simulink model "TB24_StageA_ModuleFault"  (R2025a)
settings: Solver=FixedStepDiscrete  StartTime=0  StopTime=TB.t_end  FixedStep=TB.dt  RelTol=1e-3
InitFcn:
  | % 모델과 같은 폴더의 초기화 스크립트를 실행해 P(설계 파라미터)와 TB(시험 조건)를 만든다.
  | run(fullfile(fileparts(get_param(bdroot, 'FileName')), 'TB24_init.m'));
values from neighbouring files (symbols this model uses):
  TB = struct()    [TB24_init.m]    (also in run_TB24.m = evalin('base', 'TB'))
libraries: fl_lib x126, nesl_utility x55
(part 1 of 3)
settings Model: Creator=hj000  LastModifiedBy=hj000
settings DataIOCC: SaveOutput=off  SignalLogging=off  SaveTime=off

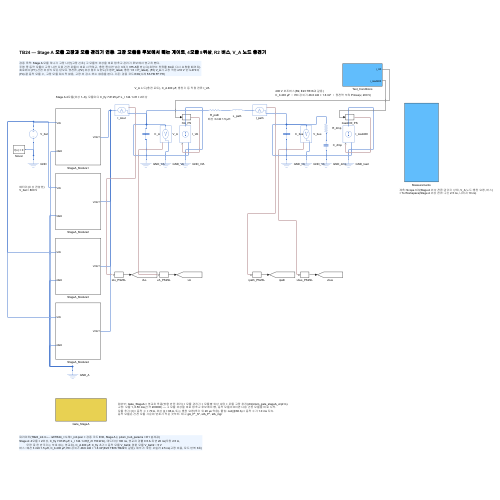
[thumbnail: Simulink's stored preview of the top-level diagram]
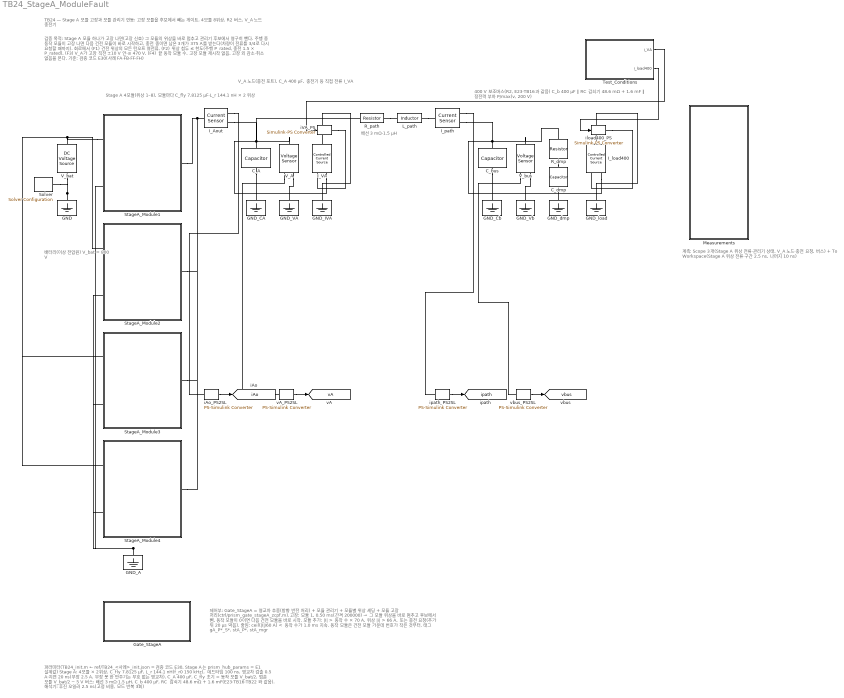
== system TB24_StageA_ModuleFault ==
  note: TB24 — Stage A 모듈 고장과 모듈 관리기 연동: 고장 모듈을 후보에서 빼는 게이트, 4모듈 8위상, R2 버스, V_A 노드 충전기
  note: 검증 목적: Stage A 모듈 하나가 고장 나면(고장 신호) 그 모듈의 위상을 바로 멈추고 관리기 후보에서 영구히 뺀다.
      | 주행 중 동작 모듈이 고장 나면 다음 건전 모듈이 바로 시작하고, 충전 중이면 남은 3개가 375 A를 받는다(차량이 전류를 3/4로 다시 요청할 때까지).
      | 회로에서 (F1) 건전 위상의 모든 턴오프 영전류, (F2) 위상 첨두 ≤ 한도(주행 P_rated, 충전 1.5 × P_rated), (F3) V_A가 고장 직전 ±10 V 안·≤ 470 V,
      | (F4) 끝 동작 모듈 수, 고장 모듈 재시작 없음, 고장 외 감소·취소 없음을 본다. 기준: 검증 코드 E30(사례 FA·FB·FF·FH)
  note: 배터리(이상 전압원)
      | V_bat = 800 V
  note: Stage A 4모듈(위상 1–8), 모듈마다 C_fly 7.8125 µF·L_r 144.1 nH × 2위상
  note: V_A 노드(충전 포트), C_A 400 µF, 충전기 등 직접 전류 I_VA
  note: 배선 3 mΩ·1.5 µH
  note: 400 V 보조버스(R2, E23·TB16과 같음)
      | C_b 400 µF ∥ RC 감쇠기 48.6 mΩ + 1.6 mF ∥ 정전력 부하 P/max(v, 200 V)
  note: 제어부: Gate_StageA = 영교차 추종(방향 반전 처리) + 모듈 관리기 + 모듈별 위상 셰딩 + 모듈 고장 처리(ctrl/prism_gate_stageA_zcpf.m).
      | 고장: 모듈 1, 0.50 ms(간격 200000) → 그 모듈 위상을 바로 멈추고 후보에서 뺌, 동작 모듈이 0이면 다음 건전 모듈을 바로 시작.
      | 모듈 추가: |I| > 동작 수 × 70 A, 위상 |i| > 66 A, 또는 충전 요청(추가 뒤 20 µs 막음). 줄임: ceil(|I|/60 A) < 동작 수가 1.0 ms 지속.
      | 동작 모듈은 건전 모듈 가운데 번호가 작은 것부터. 태그 gA_P*_S*, stA_P*, stA_mgr
  note: 계측: Scope 3개(Stage A 위상 전류·관리기 상태, V_A 노드·충전 요청, 버스)
      | + To Workspace(Stage A 위상 전류·구간 2.5 ns, 나머지 10 ns)
  note: 파라미터(TB24_init.m ← ref/TB24_<사례>_init.json = 검증 코드 E30, Stage A는 prism_hub_params = E1 설계값)
      | Stage A: 4모듈 × 2위상, C_fly 7.8125 µF, L_r 144.1 nH(f_r0 150 kHz), 데드타임 100 ns, 영교차 검출 0.5 A·지연 20 ns(무장 2.5 A,
      |          무장 못 한 반주기는 부호 없는 영교차), C_A 400 µF, C_fly 초기 = 동작 모듈 V_bat/2, 멈춘 모듈 V_bat/2 − 5 V
      | 버스: 배선 3 mΩ·1.5 µH, C_b 400 µF, RC 감쇠기 48.6 mΩ + 1.6 mF(E23·TB16·TB22와 같음). 해석기: 후진 오일러 2.5 ns(고정 비용, 모드 반복 3회)
  C_A : fl_lib/Electrical/Electrical Elements/Capacitor  c=TB.A.CA F  r=1e-6 Ohm  g=0 1/Ohm  i_specify=off  i_priority=None  i=0 A  i_nominal_specify=off  i_nominal_value=1  i_nominal_unit=A  v_specify=off  v_priority=None  v=0 V  v_nominal_specify=off  v_nominal_value=1  v_nominal_unit=V  vc_specify=on  vc_priority=High  vc=TB.vA0 V  vc_nominal_specify=off  vc_nominal_value=1  vc_nominal_unit=V
  C_bus : fl_lib/Electrical/Electrical Elements/Capacitor  c=TB.Cb F  r=1e-6 Ohm  g=0 1/Ohm  i_specify=off  i_priority=None  i=0 A  i_nominal_specify=off  i_nominal_value=1  i_nominal_unit=A  v_specify=off  v_priority=None  v=0 V  v_nominal_specify=off  v_nominal_value=1  v_nominal_unit=V  vc_specify=on  vc_priority=High  vc=TB.vb0 V  vc_nominal_specify=off  vc_nominal_value=1  vc_nominal_unit=V
  C_dmp : fl_lib/Electrical/Electrical Elements/Capacitor  c=TB.Cdmp F  r=1e-6 Ohm  g=0 1/Ohm  i_specify=off  i_priority=None  i=0 A  i_nominal_specify=off  i_nominal_value=1  i_nominal_unit=A  v_specify=off  v_priority=None  v=0 V  v_nominal_specify=off  v_nominal_value=1  v_nominal_unit=V  vc_specify=on  vc_priority=High  vc=TB.vb0 V  vc_nominal_specify=off  vc_nominal_value=1  vc_nominal_unit=V
  GND : fl_lib/Electrical/Electrical Elements/Electrical Reference
  GND_A : fl_lib/Electrical/Electrical Elements/Electrical Reference
  GND_CA : fl_lib/Electrical/Electrical Elements/Electrical Reference
  GND_Cb : fl_lib/Electrical/Electrical Elements/Electrical Reference
  GND_IVA : fl_lib/Electrical/Electrical Elements/Electrical Reference
  GND_VA : fl_lib/Electrical/Electrical Elements/Electrical Reference
  GND_Vb : fl_lib/Electrical/Electrical Elements/Electrical Reference
  GND_dmp : fl_lib/Electrical/Electrical Elements/Electrical Reference
  GND_load : fl_lib/Electrical/Electrical Elements/Electrical Reference
  Gate_StageA : Subsystem
  I_Aout : fl_lib/Electrical/Electrical Sensors/Current Sensor
  I_VA : fl_lib/Electrical/Electrical Sources/Controlled Current Source
  I_load400 : fl_lib/Electrical/Electrical Sources/Controlled Current Source
  I_path : fl_lib/Electrical/Electrical Sensors/Current Sensor
  L_path : fl_lib/Electrical/Electrical Elements/Inductor  l=TB.Lpath H  r=0 Ohm  g=1e-9 1/Ohm  i_specify=off  i_priority=None  i=0 A  i_nominal_specify=off  i_nominal_value=1  i_nominal_unit=A  v_specify=off  v_priority=None  v=0 V  v_nominal_specify=off  v_nominal_value=1  v_nominal_unit=V  i_L_specify=on  i_L_priority=High  i_L=TB.iw0 A  i_L_nominal_specify=off  i_L_nominal_value=1  i_L_nominal_unit=A
  Measurements : Subsystem
  R_dmp : fl_lib/Electrical/Electrical Elements/Resistor  R=TB.Rdmp Ohm  i_specify=off  i_priority=None  i=0 A  i_nominal_specify=off  i_nominal_value=1  i_nominal_unit=A  v_specify=off  v_priority=None  v=0 V  v_nominal_specify=off  v_nominal_value=1  v_nominal_unit=V
  R_path : fl_lib/Electrical/Electrical Elements/Resistor  R=TB.Rpath Ohm  i_specify=off  i_priority=None  i=0 A  i_nominal_specify=off  i_nominal_value=1  i_nominal_unit=A  v_specify=off  v_priority=None  v=0 V  v_nominal_specify=off  v_nominal_value=1  v_nominal_unit=V
  Solver : nesl_utility/Solver Configuration  PhysicalDomain=network_engine_domain  SubClassName=solver  LeftPortType=input  RightPortType=generic  Tones=[]  Harmonics=[]  SimulateNoise=off  Profile=off  UseLocalSampling=off  EnableSwitchedLinearOptims=on  FrequencyDomain=off  UseCCode=off  RelTol=0.001  AbsTol=0.001  MinStep=1e-09  ToWorkspace=off  RevertToSquareIcSolve=off  NumHomotopyIterations=100  PhasorMode=off  PhasorModeNumHarmonics=1  ConsistencySolver=NEWTON_XTOL_AFTER_FTOL  IndexReductionMethod=DerivativeReplacement  DoDC=off  ResidualTolerance=1e-9  ConsistencyTolSource=GLOBAL  ConsistencyAbsTol=0.001  ConsistencyRelTol=0.001  ConsistencyTolFactor=0.001  UseLocalSolver=on  LocalSolverChoice=NE_BACKWARD_EULER_ADVANCER  ResolveIndetEquations=on  FunctionEvalNumThread=1  LocalSolverSampleTime=TB.dt  DoFixedCost=on  MaxNonlinIter=3  MaxModeIter=2  ComputeImpulses=off  ImpulseIterations=2  LinearAlgebra=auto  LinearAlgebraNumThread=0  EquationFormulation=NE_TIME_EF  DelaysMemoryBudget=1024  AutomaticFiltering=on  FilteringTimeConstant=0.001  PartitionStorageMethod=AS_NEEDED  PartitionMemoryBudget=1024  PartitionMethod=ROBUST  MultibodyUseLocalSolver=off  MultibodyLocalSolverChoice=ODE1  MultibodyLocalSolverSampleTime=0.001
  StageA_Module1 : Subsystem
  StageA_Module2 : Subsystem
  StageA_Module3 : Subsystem
  StageA_Module4 : Subsystem
  Test_Conditions : Subsystem
  V_A : fl_lib/Electrical/Electrical Sensors/Voltage Sensor
  V_bat : fl_lib/Electrical/Electrical Sources/DC Voltage Source  v0=TB.vbat V
  V_bus : fl_lib/Electrical/Electrical Sensors/Voltage Sensor
  iAo_PS2SL : nesl_utility/PS-Simulink Converter  PhysicalDomain=network_engine_domain  SubClassName=ps_output  LeftPortType=input  RightPortType=output  PseudoPeriodic=off  Frequencies=[]  VectorFormat=inherit  Unit=inherit  AffineConversion=off
  iVA_PS : nesl_utility/Simulink-PS Converter  PhysicalDomain=network_engine_domain  SubClassName=ps_input  LeftPortType=input  RightPortType=output  PseudoPeriodic=off  Frequencies=[]  NoiseDistribution=none  NoiseParameters=[]  Unit=1  AffineConversion=off  FilteringAndDerivatives=provide  SimscapeFilterOrder=1  InputFilterTimeConstant=0.001  UdotUserProvided=0
  iload400_PS : nesl_utility/Simulink-PS Converter  PhysicalDomain=network_engine_domain  SubClassName=ps_input  LeftPortType=input  RightPortType=output  PseudoPeriodic=off  Frequencies=[]  NoiseDistribution=none  NoiseParameters=[]  Unit=1  AffineConversion=off  FilteringAndDerivatives=provide  SimscapeFilterOrder=1  InputFilterTimeConstant=0.001  UdotUserProvided=0
  ipath_PS2SL : nesl_utility/PS-Simulink Converter  PhysicalDomain=network_engine_domain  SubClassName=ps_output  LeftPortType=input  RightPortType=output  PseudoPeriodic=off  Frequencies=[]  VectorFormat=inherit  Unit=inherit  AffineConversion=off
  vA_PS2SL : nesl_utility/PS-Simulink Converter  PhysicalDomain=network_engine_domain  SubClassName=ps_output  LeftPortType=input  RightPortType=output  PseudoPeriodic=off  Frequencies=[]  VectorFormat=inherit  Unit=inherit  AffineConversion=off
  vbus_PS2SL : nesl_utility/PS-Simulink Converter  PhysicalDomain=network_engine_domain  SubClassName=ps_output  LeftPortType=input  RightPortType=output  PseudoPeriodic=off  Frequencies=[]  VectorFormat=inherit  Unit=inherit  AffineConversion=off
  tag scope: iAo=global, ipath=global, vA=global, vbus=global
  wires:
  iAo_PS2SL/1 -> [iAo]
  vA_PS2SL/1 -> [vA]
  ipath_PS2SL/1 -> [ipath]
  vbus_PS2SL/1 -> [vbus]
  Test_Conditions/1(i_VA) -> iVA_PS/1
  Test_Conditions/2(i_load400) -> iload400_PS/1
  connections:
  GND/LConn1 -- Solver/RConn1 -- V_bat/RConn1
  StageA_Module1/LConn1 -- V_bat/LConn1 -- StageA_Module2/LConn1 -- StageA_Module3/LConn1 -- StageA_Module4/LConn1
  StageA_Module1/LConn2 -- StageA_Module2/LConn2 -- StageA_Module3/LConn2 -- GND_A/LConn1 -- StageA_Module4/LConn2
  StageA_Module1/RConn1 -- StageA_Module2/RConn1 -- StageA_Module3/RConn1 -- I_Aout/LConn1 -- StageA_Module4/RConn1
  I_Aout/RConn2 -- V_A/LConn1 -- I_VA/RConn2 -- C_A/LConn1 -- R_path/LConn1
  C_A/RConn1 -- GND_CA/LConn1
  V_A/RConn2 -- GND_VA/LConn1
  I_VA/LConn1 -- GND_IVA/LConn1
  iVA_PS/RConn1 -- I_VA/RConn1
  R_path/RConn1 -- L_path/LConn1
  L_path/RConn1 -- I_path/LConn1
  I_path/RConn2 -- V_bus/LConn1 -- R_dmp/LConn1 -- C_bus/LConn1 -- I_load400/RConn2
  C_bus/RConn1 -- GND_Cb/LConn1
  V_bus/RConn2 -- GND_Vb/LConn1
  R_dmp/RConn1 -- C_dmp/LConn1
  C_dmp/RConn1 -- GND_dmp/LConn1
  I_load400/LConn1 -- GND_load/LConn1
  iload400_PS/RConn1 -- I_load400/RConn1
  I_Aout/RConn1 -- iAo_PS2SL/LConn1
  V_A/RConn1 -- vA_PS2SL/LConn1
  I_path/RConn1 -- ipath_PS2SL/LConn1
  V_bus/RConn1 -- vbus_PS2SL/LConn1

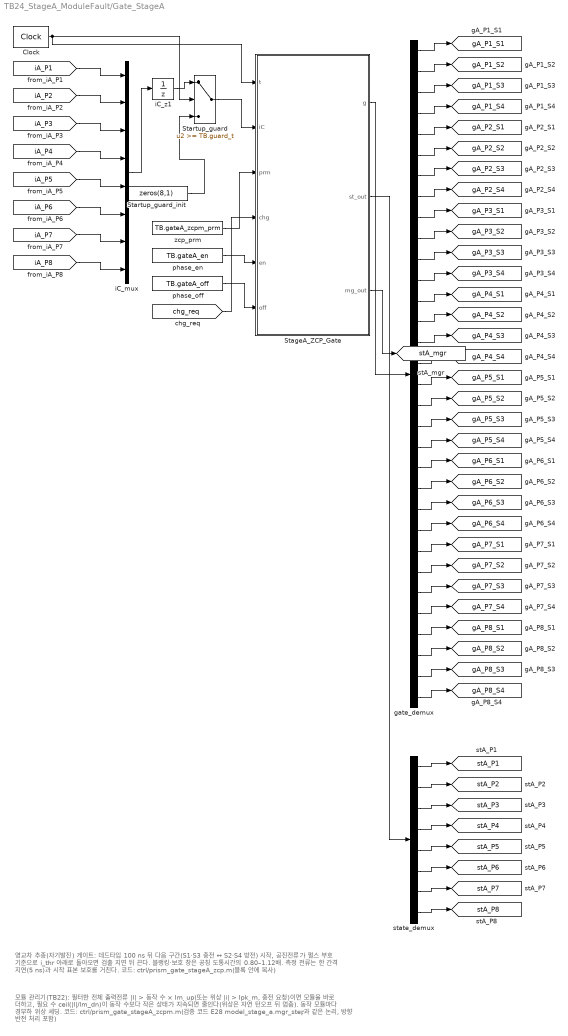
== system TB24_StageA_ModuleFault/Gate_StageA ==
  note: 모듈 관리기(TB22): 필터한 전체 출력전류 |I| > 동작 수 × Im_up(또는 위상 |i| > Ipk_m, 충전 요청)이면 모듈을 바로 더하고,
      | 필요 수 ceil(|I|/Im_dn)이 동작 수보다 작은 상태가 지속되면 줄인다(위상은 자연 턴오프 뒤 멈춤). 동작 모듈마다 경부하 위상 셰딩.
      | 코드: ctrl/prism_gate_stageA_zcpm.m(검증 코드 E28 model_stage_a.mgr_step과 같은 논리, 방향 반전 처리 포함)
  note: 영교차 추종(자기발진) 게이트: 데드타임 100 ns 뒤 다음 구간(S1·S3 충전 ↔ S2·S4 방전) 시작,
      | 공진전류가 펄스 부호 기준으로 i_thr 아래로 돌아오면 검출 지연 뒤 끈다. 블랭킹·보호 창은 공칭 도통시간의 0.80–1.12배.
      | 측정 전류는 한 간격 지연(5 ns)과 시작 표본 보호를 거친다. 코드: ctrl/prism_gate_stageA_zcp.m(블록 안에 복사)
  Clock : DigitalClock  SampleTime=TB.dt
  StageA_ZCP_Gate : MATLAB Function  TreatAsAtomicUnit=on
  Startup_guard : Switch  Threshold=TB.guard_t  SaturateOnIntegerOverflow=off  InputSameDT=off
  Startup_guard_init : Constant  Value=zeros(8,1)
  gate_demux : Demux  Outputs=[1 1 1 1 1 1 1 1 1 1 1 1 1 1 1 1 1 1 1 1 1 1 1 1 1 1 1 1 1 1 1 1]
  iC_mux : Mux  Inputs=8
  iC_z1 : UnitDelay  SampleTime=TB.dt  HasFrameUpgradeWarning=on
  phase_en : Constant  Value=TB.gateA_en
  phase_off : Constant  Value=TB.gateA_off
  state_demux : Demux  Outputs=[1 1 1 1 1 1 1 1]
  zcp_prm : Constant  Value=TB.gateA_zcpm_prm
  tag scope: gA_P1_S1=global, gA_P1_S2=global, gA_P1_S3=global, gA_P1_S4=global, gA_P2_S1=global, gA_P2_S2=global, gA_P2_S3=global, gA_P2_S4=global, gA_P3_S1=global, gA_P3_S2=global, gA_P3_S3=global, gA_P3_S4=global, gA_P4_S1=global, gA_P4_S2=global, gA_P4_S3=global, gA_P4_S4=global, gA_P5_S1=global, gA_P5_S2=global, gA_P5_S3=global, gA_P5_S4=global, gA_P6_S1=global, gA_P6_S2=global, gA_P6_S3=global, gA_P6_S4=global, gA_P7_S1=global, gA_P7_S2=global, gA_P7_S3=global, gA_P7_S4=global, gA_P8_S1=global, gA_P8_S2=global, gA_P8_S3=global, gA_P8_S4=global, stA_P1=global, stA_P2=global, stA_P3=global, stA_P4=global, stA_P5=global, stA_P6=global, stA_P7=global, stA_P8=global, stA_mgr=global
  wires:
  [iA_P1] -> iC_mux/1
  [iA_P2] -> iC_mux/2
  [iA_P3] -> iC_mux/3
  [iA_P4] -> iC_mux/4
  [iA_P5] -> iC_mux/5
  [iA_P6] -> iC_mux/6
  [iA_P7] -> iC_mux/7
  [iA_P8] -> iC_mux/8
  iC_mux/1 -> iC_z1/1
  Startup_guard_init/1 -> Startup_guard/3
  iC_z1/1 -> Startup_guard/1
  Clock/1 -> Startup_guard/2, StageA_ZCP_Gate/1(t)
  StageA_ZCP_Gate/3(mg_out) -> [stA_mgr]
  Startup_guard/1 -> StageA_ZCP_Gate/2(iC)
  zcp_prm/1 -> StageA_ZCP_Gate/3(prm)
  [chg_req] -> StageA_ZCP_Gate/4(chg)
  phase_en/1 -> StageA_ZCP_Gate/5(en)
  phase_off/1 -> StageA_ZCP_Gate/6(off)
  StageA_ZCP_Gate/1(g) -> gate_demux/1
  gate_demux/1 -> [gA_P1_S1]
  gate_demux/2 -> [gA_P1_S2]
  gate_demux/3 -> [gA_P1_S3]
  gate_demux/4 -> [gA_P1_S4]
  gate_demux/5 -> [gA_P2_S1]
  gate_demux/6 -> [gA_P2_S2]
  gate_demux/7 -> [gA_P2_S3]
  gate_demux/8 -> [gA_P2_S4]
  gate_demux/9 -> [gA_P3_S1]
  gate_demux/10 -> [gA_P3_S2]
  gate_demux/11 -> [gA_P3_S3]
  gate_demux/12 -> [gA_P3_S4]
  gate_demux/13 -> [gA_P4_S1]
  gate_demux/14 -> [gA_P4_S2]
  gate_demux/15 -> [gA_P4_S3]
  gate_demux/16 -> [gA_P4_S4]
  gate_demux/17 -> [gA_P5_S1]
  gate_demux/18 -> [gA_P5_S2]
  gate_demux/19 -> [gA_P5_S3]
  gate_demux/20 -> [gA_P5_S4]
  gate_demux/21 -> [gA_P6_S1]
  gate_demux/22 -> [gA_P6_S2]
  gate_demux/23 -> [gA_P6_S3]
  gate_demux/24 -> [gA_P6_S4]
  gate_demux/25 -> [gA_P7_S1]
  gate_demux/26 -> [gA_P7_S2]
  gate_demux/27 -> [gA_P7_S3]
  gate_demux/28 -> [gA_P7_S4]
  gate_demux/29 -> [gA_P8_S1]
  gate_demux/30 -> [gA_P8_S2]
  gate_demux/31 -> [gA_P8_S3]
  gate_demux/32 -> [gA_P8_S4]
  StageA_ZCP_Gate/2(st_out) -> state_demux/1
  state_demux/1 -> [stA_P1]
  state_demux/2 -> [stA_P2]
  state_demux/3 -> [stA_P3]
  state_demux/4 -> [stA_P4]
  state_demux/5 -> [stA_P5]
  state_demux/6 -> [stA_P6]
  state_demux/7 -> [stA_P7]
  state_demux/8 -> [stA_P8]

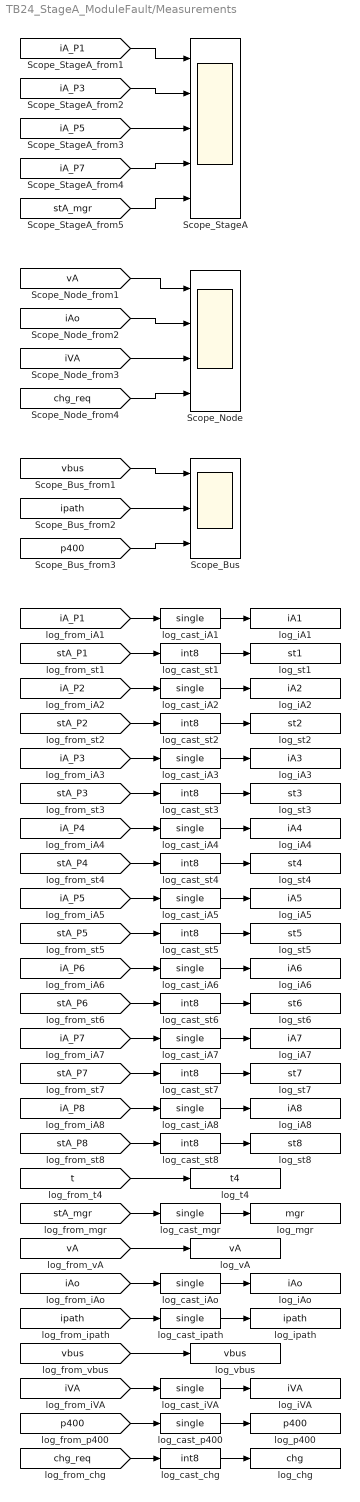
== system TB24_StageA_ModuleFault/Measurements ==
  Scope_Bus : Scope  NumInputPorts=3
      settings: Title=Scope Bus
  Scope_Node : Scope  NumInputPorts=4
      settings: Title=Scope Node
  Scope_StageA : Scope  NumInputPorts=5
      settings: Title=Scope StageA
  log_cast_chg : DataTypeConversion  OutDataTypeStr=int8  SaturateOnIntegerOverflow=off  RndMeth=Floor
  log_cast_iA{1..8} (8 alike) : DataTypeConversion  OutDataTypeStr=single  SaturateOnIntegerOverflow=off  RndMeth=Floor
  log_cast_iAo : DataTypeConversion  OutDataTypeStr=single  SaturateOnIntegerOverflow=off  RndMeth=Floor
  log_cast_iVA : DataTypeConversion  OutDataTypeStr=single  SaturateOnIntegerOverflow=off  RndMeth=Floor
  log_cast_ipath : DataTypeConversion  OutDataTypeStr=single  SaturateOnIntegerOverflow=off  RndMeth=Floor
  log_cast_mgr : DataTypeConversion  OutDataTypeStr=single  SaturateOnIntegerOverflow=off  RndMeth=Floor
  log_cast_p400 : DataTypeConversion  OutDataTypeStr=single  SaturateOnIntegerOverflow=off  RndMeth=Floor
  log_cast_st{1..8} (8 alike) : DataTypeConversion  OutDataTypeStr=int8  SaturateOnIntegerOverflow=off  RndMeth=Floor
  log_chg : ToWorkspace  VariableName=chg  SampleTime=-1
      settings: Decimation=4
  log_iA1 : ToWorkspace  VariableName=iA1  SampleTime=-1
  log_iA2 : ToWorkspace  VariableName=iA2  SampleTime=-1
  log_iA3 : ToWorkspace  VariableName=iA3  SampleTime=-1
  log_iA4 : ToWorkspace  VariableName=iA4  SampleTime=-1
  log_iA5 : ToWorkspace  VariableName=iA5  SampleTime=-1
  log_iA6 : ToWorkspace  VariableName=iA6  SampleTime=-1
  log_iA7 : ToWorkspace  VariableName=iA7  SampleTime=-1
  log_iA8 : ToWorkspace  VariableName=iA8  SampleTime=-1
  log_iAo : ToWorkspace  VariableName=iAo  SampleTime=-1
      settings: Decimation=4
  log_iVA : ToWorkspace  VariableName=iVA  SampleTime=-1
      settings: Decimation=4
  log_ipath : ToWorkspace  VariableName=ipath  SampleTime=-1
      settings: Decimation=4
  log_mgr : ToWorkspace  VariableName=mgr  SampleTime=-1
      settings: Decimation=4
  log_p400 : ToWorkspace  VariableName=p400  SampleTime=-1
      settings: Decimation=4
  log_st1 : ToWorkspace  VariableName=st1  SampleTime=-1
  log_st2 : ToWorkspace  VariableName=st2  SampleTime=-1
  log_st3 : ToWorkspace  VariableName=st3  SampleTime=-1
  log_st4 : ToWorkspace  VariableName=st4  SampleTime=-1
  log_st5 : ToWorkspace  VariableName=st5  SampleTime=-1
  log_st6 : ToWorkspace  VariableName=st6  SampleTime=-1
  log_st7 : ToWorkspace  VariableName=st7  SampleTime=-1
  log_st8 : ToWorkspace  VariableName=st8  SampleTime=-1
  log_t4 : ToWorkspace  VariableName=t4  SampleTime=-1
      settings: Decimation=4
  log_vA : ToWorkspace  VariableName=vA  SampleTime=-1
      settings: Decimation=4
  log_vbus : ToWorkspace  VariableName=vbus  SampleTime=-1
      settings: Decimation=4
  wires:
  [iA_P1] -> Scope_StageA/1
  [iA_P3] -> Scope_StageA/2
  [iA_P5] -> Scope_StageA/3
  [iA_P7] -> Scope_StageA/4
  [stA_mgr] -> Scope_StageA/5
  [vA] -> Scope_Node/1
  [iAo] -> Scope_Node/2
  [iVA] -> Scope_Node/3
  [chg_req] -> Scope_Node/4
  [vbus] -> Scope_Bus/1
  [ipath] -> Scope_Bus/2
  [p400] -> Scope_Bus/3
  [iA_P1] -> log_cast_iA1/1
  log_cast_iA1/1 -> log_iA1/1
  [stA_P1] -> log_cast_st1/1
  log_cast_st1/1 -> log_st1/1
  [iA_P2] -> log_cast_iA2/1
  log_cast_iA2/1 -> log_iA2/1
  [stA_P2] -> log_cast_st2/1
  log_cast_st2/1 -> log_st2/1
  [iA_P3] -> log_cast_iA3/1
  log_cast_iA3/1 -> log_iA3/1
  [stA_P3] -> log_cast_st3/1
  log_cast_st3/1 -> log_st3/1
  [iA_P4] -> log_cast_iA4/1
  log_cast_iA4/1 -> log_iA4/1
  [stA_P4] -> log_cast_st4/1
  log_cast_st4/1 -> log_st4/1
  [iA_P5] -> log_cast_iA5/1
  log_cast_iA5/1 -> log_iA5/1
  [stA_P5] -> log_cast_st5/1
  log_cast_st5/1 -> log_st5/1
  [iA_P6] -> log_cast_iA6/1
  log_cast_iA6/1 -> log_iA6/1
  [stA_P6] -> log_cast_st6/1
  log_cast_st6/1 -> log_st6/1
  [iA_P7] -> log_cast_iA7/1
  log_cast_iA7/1 -> log_iA7/1
  [stA_P7] -> log_cast_st7/1
  log_cast_st7/1 -> log_st7/1
  [iA_P8] -> log_cast_iA8/1
  log_cast_iA8/1 -> log_iA8/1
  [stA_P8] -> log_cast_st8/1
  log_cast_st8/1 -> log_st8/1
  [t] -> log_t4/1
  [stA_mgr] -> log_cast_mgr/1
  log_cast_mgr/1 -> log_mgr/1
  [vA] -> log_vA/1
  [iAo] -> log_cast_iAo/1
  log_cast_iAo/1 -> log_iAo/1
  [ipath] -> log_cast_ipath/1
  log_cast_ipath/1 -> log_ipath/1
  [vbus] -> log_vbus/1
  [iVA] -> log_cast_iVA/1
  log_cast_iVA/1 -> log_iVA/1
  [p400] -> log_cast_p400/1
  log_cast_p400/1 -> log_p400/1
  [chg_req] -> log_cast_chg/1
  log_cast_chg/1 -> log_chg/1

== system TB24_StageA_ModuleFault/StageA_Module1 ==
  note: Stage A 모듈 1: 위상 1·2 병렬(목표 정격 37.5 kW)
      | 각 위상은 영교차 추종 게이트로 자기 공진전류가 0일 때 끈다(ZCS). 두 위상은 T/4 엇갈려 시작한다.
  StageA_Phase1 : Subsystem
  StageA_Phase2 : Subsystem
  VIN : PMIOPort  Side=Left
  GND : PMIOPort  Port=2  Side=Left
  VOUT : PMIOPort  Port=3  Side=Right
  connections:
  VIN/RConn1 -- StageA_Phase1/LConn1 -- StageA_Phase2/LConn1
  GND/RConn1 -- StageA_Phase1/LConn2 -- StageA_Phase2/LConn2
  VOUT/RConn1 -- StageA_Phase1/RConn1 -- StageA_Phase2/RConn1

== system TB24_StageA_ModuleFault/StageA_Module2 ==
  note: Stage A 모듈 2: 위상 3·4 병렬(목표 정격 37.5 kW)
      | 각 위상은 영교차 추종 게이트로 자기 공진전류가 0일 때 끈다(ZCS). 두 위상은 T/4 엇갈려 시작한다.
  StageA_Phase3 : Subsystem
  StageA_Phase4 : Subsystem
  VIN : PMIOPort  Side=Left
  GND : PMIOPort  Port=2  Side=Left
  VOUT : PMIOPort  Port=3  Side=Right
  connections:
  VIN/RConn1 -- StageA_Phase3/LConn1 -- StageA_Phase4/LConn1
  GND/RConn1 -- StageA_Phase3/LConn2 -- StageA_Phase4/LConn2
  VOUT/RConn1 -- StageA_Phase3/RConn1 -- StageA_Phase4/RConn1

== system TB24_StageA_ModuleFault/StageA_Module3 ==
  note: Stage A 모듈 3: 위상 5·6 병렬(목표 정격 37.5 kW)
      | 각 위상은 영교차 추종 게이트로 자기 공진전류가 0일 때 끈다(ZCS). 두 위상은 T/4 엇갈려 시작한다.
  StageA_Phase5 : Subsystem
  StageA_Phase6 : Subsystem
  VIN : PMIOPort  Side=Left
  GND : PMIOPort  Port=2  Side=Left
  VOUT : PMIOPort  Port=3  Side=Right
  connections:
  VIN/RConn1 -- StageA_Phase5/LConn1 -- StageA_Phase6/LConn1
  GND/RConn1 -- StageA_Phase5/LConn2 -- StageA_Phase6/LConn2
  VOUT/RConn1 -- StageA_Phase5/RConn1 -- StageA_Phase6/RConn1

== system TB24_StageA_ModuleFault/StageA_Module4 ==
  note: Stage A 모듈 4: 위상 7·8 병렬(목표 정격 37.5 kW)
      | 각 위상은 영교차 추종 게이트로 자기 공진전류가 0일 때 끈다(ZCS). 두 위상은 T/4 엇갈려 시작한다.
  StageA_Phase7 : Subsystem
  StageA_Phase8 : Subsystem
  VIN : PMIOPort  Side=Left
  GND : PMIOPort  Port=2  Side=Left
  VOUT : PMIOPort  Port=3  Side=Right
  connections:
  VIN/RConn1 -- StageA_Phase7/LConn1 -- StageA_Phase8/LConn1
  GND/RConn1 -- StageA_Phase7/LConn2 -- StageA_Phase8/LConn2
  VOUT/RConn1 -- StageA_Phase7/RConn1 -- StageA_Phase8/RConn1

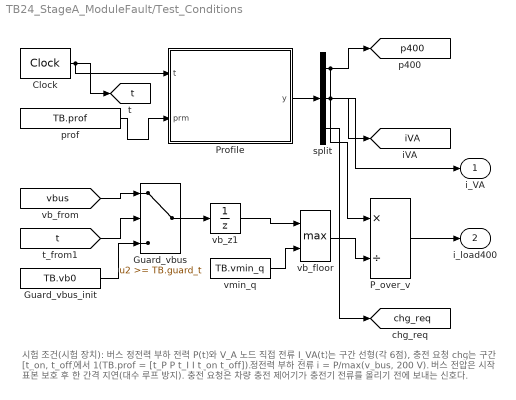
== system TB24_StageA_ModuleFault/Test_Conditions ==
  note: 시험 조건(시험 장치): 버스 정전력 부하 전력 P(t)와 V_A 노드 직접 전류 I_VA(t)는 구간 선형(각 6점), 충전 요청 chg는 구간
      | [t_on, t_off)에서 1(TB.prof = [t_P P t_I I t_on t_off]). 정전력 부하 전류 i = P/max(v_bus, 200 V). 버스 전압은 시작 표본 보호 후
      | 한 간격 지연(대수 루프 방지). 충전 요청은 차량 충전 제어기가 충전기 전류를 올리기 전에 보내는 신호다.
  Clock : DigitalClock  SampleTime=TB.dt
  Guard_vbus : Switch  Threshold=TB.guard_t  SaturateOnIntegerOverflow=off  InputSameDT=off
  Guard_vbus_init : Constant  Value=TB.vb0
  P_over_v : Product  Inputs=*/
  Profile : MATLAB Function  TreatAsAtomicUnit=on
  prof : Constant  Value=TB.prof
  split : Demux  Outputs=3
  vb_floor : MinMax  Function=max  Inputs=2
  vb_z1 : UnitDelay  SampleTime=TB.dt  HasFrameUpgradeWarning=on
  vmin_q : Constant  Value=TB.vmin_q
  i_VA : Outport
  i_load400 : Outport  Port=2
  tag scope: chg_req=global, iVA=global, p400=global, t=global
  wires:
  Clock/1 -> [t], Profile/1(t)
  prof/1 -> Profile/2(prm)
  Profile/1(y) -> split/1
  split/1 -> [p400], P_over_v/1
  split/2 -> [iVA], i_VA/1
  split/3 -> [chg_req]
  Guard_vbus_init/1 -> Guard_vbus/3
  [vbus] -> Guard_vbus/1
  [t] -> Guard_vbus/2
  Guard_vbus/1 -> vb_z1/1
  vb_z1/1 -> vb_floor/1
  vmin_q/1 -> vb_floor/2
  vb_floor/1 -> P_over_v/2
  P_over_v/1 -> i_load400/1

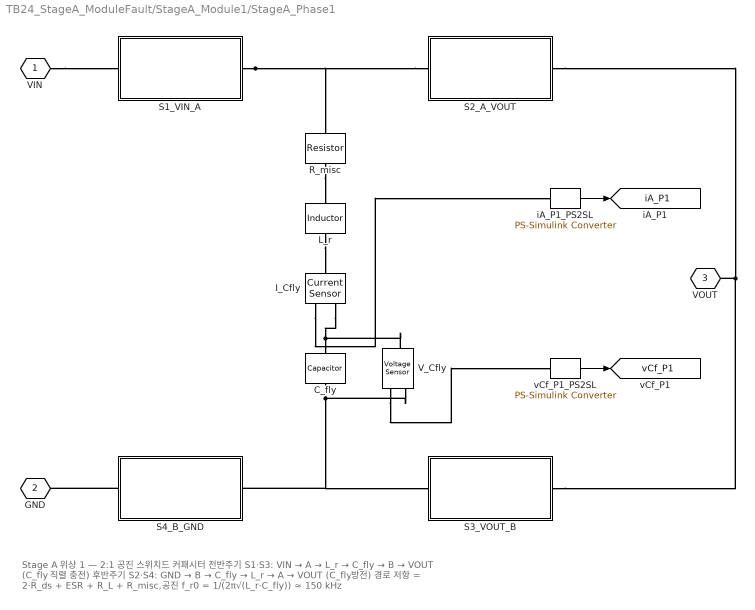
== system TB24_StageA_ModuleFault/StageA_Module1/StageA_Phase1 ==
  note: Stage A 위상 1 — 2:1 공진 스위치드 커패시터
      | 전반주기 S1·S3: VIN → A → L_r → C_fly → B → VOUT (C_fly 직렬 충전)
      | 후반주기 S2·S4: GND → B → C_fly → L_r → A → VOUT (C_fly 방전)
      | 경로 저항 = 2·R_ds + ESR + R_L + R_misc, 공진 f_r0 = 1/(2π√(L_r·C_fly)) ≈ 150 kHz
  C_fly : fl_lib/Electrical/Electrical Elements/Capacitor  c=TB.A.Cfly F  r=TB.A.ESR Ohm  g=0 1/Ohm  i_specify=off  i_priority=None  i=0 A  i_nominal_specify=off  i_nominal_value=1  i_nominal_unit=A  v_specify=off  v_priority=None  v=0 V  v_nominal_specify=off  v_nominal_value=1  v_nominal_unit=V  vc_specify=on  vc_priority=High  vc=TB.vC0_ph(1) V  vc_nominal_specify=off  vc_nominal_value=1  vc_nominal_unit=V
  I_Cfly : fl_lib/Electrical/Electrical Sensors/Current Sensor
  L_r : fl_lib/Electrical/Electrical Elements/Inductor  l=TB.A.Lr H  r=TB.A.RL Ohm  g=1e-9 1/Ohm  i_specify=off  i_priority=None  i=0 A  i_nominal_specify=off  i_nominal_value=1  i_nominal_unit=A  v_specify=off  v_priority=None  v=0 V  v_nominal_specify=off  v_nominal_value=1  v_nominal_unit=V  i_L_specify=on  i_L_priority=High  i_L=0 A  i_L_nominal_specify=off  i_L_nominal_value=1  i_L_nominal_unit=A
  R_misc : fl_lib/Electrical/Electrical Elements/Resistor  R=TB.A.Rmisc Ohm  i_specify=off  i_priority=None  i=0 A  i_nominal_specify=off  i_nominal_value=1  i_nominal_unit=A  v_specify=off  v_priority=None  v=0 V  v_nominal_specify=off  v_nominal_value=1  v_nominal_unit=V
  S1_VIN_A : Subsystem  mask(PRISM-Hub switch cell){Ron=TB.A.Rds, Goff=TB.A.Goff, Vf=TB.A.Vf, Rd=TB.A.Rd, Goffd=TB.A.Goffd}
      mask prompts: Ron "도통 저항 R_on [Ohm]"; Goff "차단 컨덕턴스 G_off [S]"; Vf "다이오드 순방향 전압 Vf [V]"; Rd "다이오드 도통 저항 R_d [Ohm]"; Goffd "다이오드 차단 컨덕턴스 [S]"
      mask help: 전력 반도체 스위치 셀 S1. 게이트 태그 gA_P1_S1.
      settings: AttributesFormatString=gate: gA_P1_S1
      mask Display:
      | plot([0.05 0.35 ],[0.50 0.50 ],[0.35 0.65 ],[0.50 0.74 ],[0.65 0.95 ],[0.50 0.50 ]);
      | plot([0.20 0.20 0.42 ],[0.50 0.20 0.20 ],[0.58 0.80 0.80 ],[0.20 0.20 0.50 ]);
      | plot([0.42 0.58 0.58 0.42 ],[0.20 0.10 0.30 0.20 ],[0.42 0.42 ],[0.10 0.30 ]);
      | text(0.5,0.80,'S1','horizontalAlignment','center','texmode','off');
      | port_label('LConn',1,'D');
      | port_label('RConn',1,'S');
  S2_A_VOUT : Subsystem  mask(PRISM-Hub switch cell){Ron=TB.A.Rds, Goff=TB.A.Goff, Vf=TB.A.Vf, Rd=TB.A.Rd, Goffd=TB.A.Goffd}
      mask prompts: Ron "도통 저항 R_on [Ohm]"; Goff "차단 컨덕턴스 G_off [S]"; Vf "다이오드 순방향 전압 Vf [V]"; Rd "다이오드 도통 저항 R_d [Ohm]"; Goffd "다이오드 차단 컨덕턴스 [S]"
      mask help: 전력 반도체 스위치 셀 S2. 게이트 태그 gA_P1_S2.
      settings: AttributesFormatString=gate: gA_P1_S2
      mask Display:
      | plot([0.05 0.35 ],[0.50 0.50 ],[0.35 0.65 ],[0.50 0.74 ],[0.65 0.95 ],[0.50 0.50 ]);
      | plot([0.20 0.20 0.42 ],[0.50 0.20 0.20 ],[0.58 0.80 0.80 ],[0.20 0.20 0.50 ]);
      | plot([0.42 0.58 0.58 0.42 ],[0.20 0.10 0.30 0.20 ],[0.42 0.42 ],[0.10 0.30 ]);
      | text(0.5,0.80,'S2','horizontalAlignment','center','texmode','off');
      | port_label('LConn',1,'D');
      | port_label('RConn',1,'S');
  S3_VOUT_B : Subsystem  mask(PRISM-Hub switch cell){Ron=TB.A.Rds, Goff=TB.A.Goff, Vf=TB.A.Vf, Rd=TB.A.Rd, Goffd=TB.A.Goffd}
      mask prompts: Ron "도통 저항 R_on [Ohm]"; Goff "차단 컨덕턴스 G_off [S]"; Vf "다이오드 순방향 전압 Vf [V]"; Rd "다이오드 도통 저항 R_d [Ohm]"; Goffd "다이오드 차단 컨덕턴스 [S]"
      mask help: 전력 반도체 스위치 셀 S3. 게이트 태그 gA_P1_S3.
      settings: AttributesFormatString=gate: gA_P1_S3
      mask Display:
      | plot([0.95 0.65 ],[0.50 0.50 ],[0.65 0.35 ],[0.50 0.74 ],[0.35 0.05 ],[0.50 0.50 ]);
      | plot([0.80 0.80 0.58 ],[0.50 0.20 0.20 ],[0.42 0.20 0.20 ],[0.20 0.20 0.50 ]);
      | plot([0.58 0.42 0.42 0.58 ],[0.20 0.10 0.30 0.20 ],[0.58 0.58 ],[0.10 0.30 ]);
      | text(0.5,0.80,'S3','horizontalAlignment','center','texmode','off');
      | port_label('LConn',1,'D');
      | port_label('RConn',1,'S');
  S4_B_GND : Subsystem  mask(PRISM-Hub switch cell){Ron=TB.A.Rds, Goff=TB.A.Goff, Vf=TB.A.Vf, Rd=TB.A.Rd, Goffd=TB.A.Goffd}
      mask prompts: Ron "도통 저항 R_on [Ohm]"; Goff "차단 컨덕턴스 G_off [S]"; Vf "다이오드 순방향 전압 Vf [V]"; Rd "다이오드 도통 저항 R_d [Ohm]"; Goffd "다이오드 차단 컨덕턴스 [S]"
      mask help: 전력 반도체 스위치 셀 S4. 게이트 태그 gA_P1_S4.
      settings: AttributesFormatString=gate: gA_P1_S4
      mask Display:
      | plot([0.95 0.65 ],[0.50 0.50 ],[0.65 0.35 ],[0.50 0.74 ],[0.35 0.05 ],[0.50 0.50 ]);
      | plot([0.80 0.80 0.58 ],[0.50 0.20 0.20 ],[0.42 0.20 0.20 ],[0.20 0.20 0.50 ]);
      | plot([0.58 0.42 0.42 0.58 ],[0.20 0.10 0.30 0.20 ],[0.58 0.58 ],[0.10 0.30 ]);
      | text(0.5,0.80,'S4','horizontalAlignment','center','texmode','off');
      | port_label('LConn',1,'D');
      | port_label('RConn',1,'S');
  V_Cfly : fl_lib/Electrical/Electrical Sensors/Voltage Sensor
  iA_P1_PS2SL : nesl_utility/PS-Simulink Converter  PhysicalDomain=network_engine_domain  SubClassName=ps_output  LeftPortType=input  RightPortType=output  PseudoPeriodic=off  Frequencies=[]  VectorFormat=inherit  Unit=inherit  AffineConversion=off
  vCf_P1_PS2SL : nesl_utility/PS-Simulink Converter  PhysicalDomain=network_engine_domain  SubClassName=ps_output  LeftPortType=input  RightPortType=output  PseudoPeriodic=off  Frequencies=[]  VectorFormat=inherit  Unit=inherit  AffineConversion=off
  VIN : PMIOPort  Side=Left
  GND : PMIOPort  Port=2  Side=Left
  VOUT : PMIOPort  Port=3  Side=Right
  tag scope: iA_P1=global, vCf_P1=global
  wires:
  iA_P1_PS2SL/1 -> [iA_P1]
  vCf_P1_PS2SL/1 -> [vCf_P1]
  connections:
  VIN/RConn1 -- S1_VIN_A/LConn1
  S2_A_VOUT/LConn1 -- S1_VIN_A/RConn1 -- R_misc/LConn1
  R_misc/RConn1 -- L_r/LConn1
  L_r/RConn1 -- I_Cfly/LConn1
  C_fly/LConn1 -- I_Cfly/RConn2 -- V_Cfly/LConn1
  S4_B_GND/LConn1 -- C_fly/RConn1 -- S3_VOUT_B/RConn1 -- V_Cfly/RConn2
  S4_B_GND/RConn1 -- GND/RConn1
  VOUT/RConn1 -- S2_A_VOUT/RConn1 -- S3_VOUT_B/LConn1
  I_Cfly/RConn1 -- iA_P1_PS2SL/LConn1
  V_Cfly/RConn1 -- vCf_P1_PS2SL/LConn1

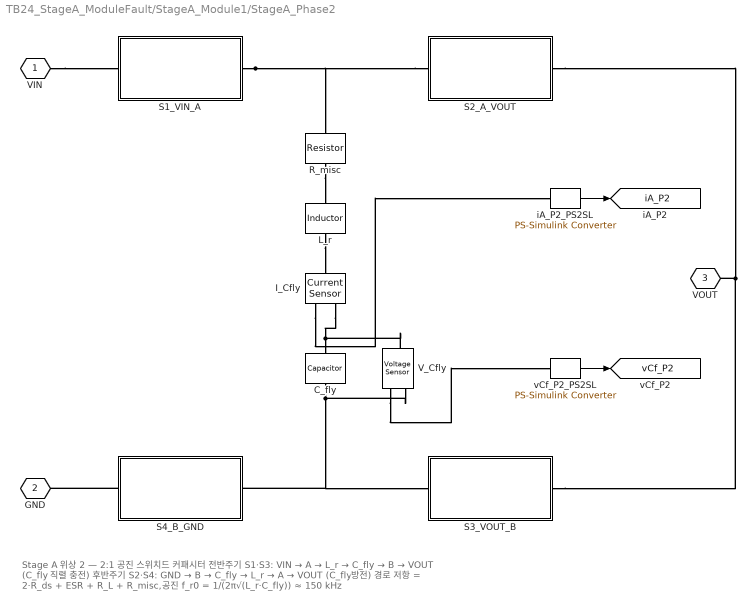
== system TB24_StageA_ModuleFault/StageA_Module1/StageA_Phase2 ==
  note: Stage A 위상 2 — 2:1 공진 스위치드 커패시터
      | 전반주기 S1·S3: VIN → A → L_r → C_fly → B → VOUT (C_fly 직렬 충전)
      | 후반주기 S2·S4: GND → B → C_fly → L_r → A → VOUT (C_fly 방전)
      | 경로 저항 = 2·R_ds + ESR + R_L + R_misc, 공진 f_r0 = 1/(2π√(L_r·C_fly)) ≈ 150 kHz
  C_fly : fl_lib/Electrical/Electrical Elements/Capacitor  c=TB.A.Cfly F  r=TB.A.ESR Ohm  g=0 1/Ohm  i_specify=off  i_priority=None  i=0 A  i_nominal_specify=off  i_nominal_value=1  i_nominal_unit=A  v_specify=off  v_priority=None  v=0 V  v_nominal_specify=off  v_nominal_value=1  v_nominal_unit=V  vc_specify=on  vc_priority=High  vc=TB.vC0_ph(2) V  vc_nominal_specify=off  vc_nominal_value=1  vc_nominal_unit=V
  I_Cfly : fl_lib/Electrical/Electrical Sensors/Current Sensor
  L_r : fl_lib/Electrical/Electrical Elements/Inductor  l=TB.A.Lr H  r=TB.A.RL Ohm  g=1e-9 1/Ohm  i_specify=off  i_priority=None  i=0 A  i_nominal_specify=off  i_nominal_value=1  i_nominal_unit=A  v_specify=off  v_priority=None  v=0 V  v_nominal_specify=off  v_nominal_value=1  v_nominal_unit=V  i_L_specify=on  i_L_priority=High  i_L=0 A  i_L_nominal_specify=off  i_L_nominal_value=1  i_L_nominal_unit=A
  R_misc : fl_lib/Electrical/Electrical Elements/Resistor  R=TB.A.Rmisc Ohm  i_specify=off  i_priority=None  i=0 A  i_nominal_specify=off  i_nominal_value=1  i_nominal_unit=A  v_specify=off  v_priority=None  v=0 V  v_nominal_specify=off  v_nominal_value=1  v_nominal_unit=V
  S1_VIN_A : Subsystem  mask(PRISM-Hub switch cell){Ron=TB.A.Rds, Goff=TB.A.Goff, Vf=TB.A.Vf, Rd=TB.A.Rd, Goffd=TB.A.Goffd}
      mask prompts: Ron "도통 저항 R_on [Ohm]"; Goff "차단 컨덕턴스 G_off [S]"; Vf "다이오드 순방향 전압 Vf [V]"; Rd "다이오드 도통 저항 R_d [Ohm]"; Goffd "다이오드 차단 컨덕턴스 [S]"
      mask help: 전력 반도체 스위치 셀 S1. 게이트 태그 gA_P2_S1.
      settings: AttributesFormatString=gate: gA_P2_S1
      mask Display:
      | plot([0.05 0.35 ],[0.50 0.50 ],[0.35 0.65 ],[0.50 0.74 ],[0.65 0.95 ],[0.50 0.50 ]);
      | plot([0.20 0.20 0.42 ],[0.50 0.20 0.20 ],[0.58 0.80 0.80 ],[0.20 0.20 0.50 ]);
      | plot([0.42 0.58 0.58 0.42 ],[0.20 0.10 0.30 0.20 ],[0.42 0.42 ],[0.10 0.30 ]);
      | text(0.5,0.80,'S1','horizontalAlignment','center','texmode','off');
      | port_label('LConn',1,'D');
      | port_label('RConn',1,'S');
  S2_A_VOUT : Subsystem  mask(PRISM-Hub switch cell){Ron=TB.A.Rds, Goff=TB.A.Goff, Vf=TB.A.Vf, Rd=TB.A.Rd, Goffd=TB.A.Goffd}
      mask prompts: Ron "도통 저항 R_on [Ohm]"; Goff "차단 컨덕턴스 G_off [S]"; Vf "다이오드 순방향 전압 Vf [V]"; Rd "다이오드 도통 저항 R_d [Ohm]"; Goffd "다이오드 차단 컨덕턴스 [S]"
      mask help: 전력 반도체 스위치 셀 S2. 게이트 태그 gA_P2_S2.
      settings: AttributesFormatString=gate: gA_P2_S2
      mask Display:
      | plot([0.05 0.35 ],[0.50 0.50 ],[0.35 0.65 ],[0.50 0.74 ],[0.65 0.95 ],[0.50 0.50 ]);
      | plot([0.20 0.20 0.42 ],[0.50 0.20 0.20 ],[0.58 0.80 0.80 ],[0.20 0.20 0.50 ]);
      | plot([0.42 0.58 0.58 0.42 ],[0.20 0.10 0.30 0.20 ],[0.42 0.42 ],[0.10 0.30 ]);
      | text(0.5,0.80,'S2','horizontalAlignment','center','texmode','off');
      | port_label('LConn',1,'D');
      | port_label('RConn',1,'S');
  S3_VOUT_B : Subsystem  mask(PRISM-Hub switch cell){Ron=TB.A.Rds, Goff=TB.A.Goff, Vf=TB.A.Vf, Rd=TB.A.Rd, Goffd=TB.A.Goffd}
      mask prompts: Ron "도통 저항 R_on [Ohm]"; Goff "차단 컨덕턴스 G_off [S]"; Vf "다이오드 순방향 전압 Vf [V]"; Rd "다이오드 도통 저항 R_d [Ohm]"; Goffd "다이오드 차단 컨덕턴스 [S]"
      mask help: 전력 반도체 스위치 셀 S3. 게이트 태그 gA_P2_S3.
      settings: AttributesFormatString=gate: gA_P2_S3
      mask Display:
      | plot([0.95 0.65 ],[0.50 0.50 ],[0.65 0.35 ],[0.50 0.74 ],[0.35 0.05 ],[0.50 0.50 ]);
      | plot([0.80 0.80 0.58 ],[0.50 0.20 0.20 ],[0.42 0.20 0.20 ],[0.20 0.20 0.50 ]);
      | plot([0.58 0.42 0.42 0.58 ],[0.20 0.10 0.30 0.20 ],[0.58 0.58 ],[0.10 0.30 ]);
      | text(0.5,0.80,'S3','horizontalAlignment','center','texmode','off');
      | port_label('LConn',1,'D');
      | port_label('RConn',1,'S');
  S4_B_GND : Subsystem  mask(PRISM-Hub switch cell){Ron=TB.A.Rds, Goff=TB.A.Goff, Vf=TB.A.Vf, Rd=TB.A.Rd, Goffd=TB.A.Goffd}
      mask prompts: Ron "도통 저항 R_on [Ohm]"; Goff "차단 컨덕턴스 G_off [S]"; Vf "다이오드 순방향 전압 Vf [V]"; Rd "다이오드 도통 저항 R_d [Ohm]"; Goffd "다이오드 차단 컨덕턴스 [S]"
      mask help: 전력 반도체 스위치 셀 S4. 게이트 태그 gA_P2_S4.
      settings: AttributesFormatString=gate: gA_P2_S4
      mask Display:
      | plot([0.95 0.65 ],[0.50 0.50 ],[0.65 0.35 ],[0.50 0.74 ],[0.35 0.05 ],[0.50 0.50 ]);
      | plot([0.80 0.80 0.58 ],[0.50 0.20 0.20 ],[0.42 0.20 0.20 ],[0.20 0.20 0.50 ]);
      | plot([0.58 0.42 0.42 0.58 ],[0.20 0.10 0.30 0.20 ],[0.58 0.58 ],[0.10 0.30 ]);
      | text(0.5,0.80,'S4','horizontalAlignment','center','texmode','off');
      | port_label('LConn',1,'D');
      | port_label('RConn',1,'S');
  V_Cfly : fl_lib/Electrical/Electrical Sensors/Voltage Sensor
  iA_P2_PS2SL : nesl_utility/PS-Simulink Converter  PhysicalDomain=network_engine_domain  SubClassName=ps_output  LeftPortType=input  RightPortType=output  PseudoPeriodic=off  Frequencies=[]  VectorFormat=inherit  Unit=inherit  AffineConversion=off
  vCf_P2_PS2SL : nesl_utility/PS-Simulink Converter  PhysicalDomain=network_engine_domain  SubClassName=ps_output  LeftPortType=input  RightPortType=output  PseudoPeriodic=off  Frequencies=[]  VectorFormat=inherit  Unit=inherit  AffineConversion=off
  VIN : PMIOPort  Side=Left
  GND : PMIOPort  Port=2  Side=Left
  VOUT : PMIOPort  Port=3  Side=Right
  tag scope: iA_P2=global, vCf_P2=global
  wires:
  iA_P2_PS2SL/1 -> [iA_P2]
  vCf_P2_PS2SL/1 -> [vCf_P2]
  connections:
  VIN/RConn1 -- S1_VIN_A/LConn1
  S2_A_VOUT/LConn1 -- S1_VIN_A/RConn1 -- R_misc/LConn1
  R_misc/RConn1 -- L_r/LConn1
  L_r/RConn1 -- I_Cfly/LConn1
  C_fly/LConn1 -- I_Cfly/RConn2 -- V_Cfly/LConn1
  S4_B_GND/LConn1 -- C_fly/RConn1 -- S3_VOUT_B/RConn1 -- V_Cfly/RConn2
  S4_B_GND/RConn1 -- GND/RConn1
  VOUT/RConn1 -- S2_A_VOUT/RConn1 -- S3_VOUT_B/LConn1
  I_Cfly/RConn1 -- iA_P2_PS2SL/LConn1
  V_Cfly/RConn1 -- vCf_P2_PS2SL/LConn1

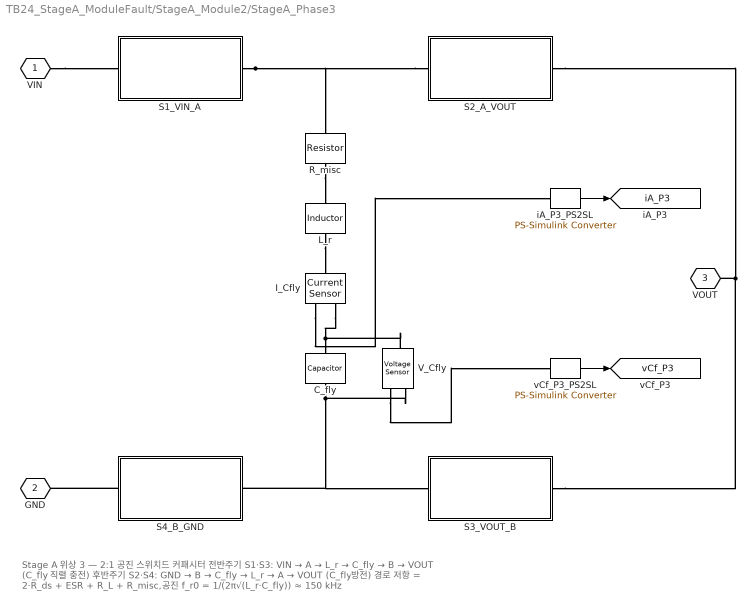
== system TB24_StageA_ModuleFault/StageA_Module2/StageA_Phase3 ==
  note: Stage A 위상 3 — 2:1 공진 스위치드 커패시터
      | 전반주기 S1·S3: VIN → A → L_r → C_fly → B → VOUT (C_fly 직렬 충전)
      | 후반주기 S2·S4: GND → B → C_fly → L_r → A → VOUT (C_fly 방전)
      | 경로 저항 = 2·R_ds + ESR + R_L + R_misc, 공진 f_r0 = 1/(2π√(L_r·C_fly)) ≈ 150 kHz
  C_fly : fl_lib/Electrical/Electrical Elements/Capacitor  c=TB.A.Cfly F  r=TB.A.ESR Ohm  g=0 1/Ohm  i_specify=off  i_priority=None  i=0 A  i_nominal_specify=off  i_nominal_value=1  i_nominal_unit=A  v_specify=off  v_priority=None  v=0 V  v_nominal_specify=off  v_nominal_value=1  v_nominal_unit=V  vc_specify=on  vc_priority=High  vc=TB.vC0_ph(3) V  vc_nominal_specify=off  vc_nominal_value=1  vc_nominal_unit=V
  I_Cfly : fl_lib/Electrical/Electrical Sensors/Current Sensor
  L_r : fl_lib/Electrical/Electrical Elements/Inductor  l=TB.A.Lr H  r=TB.A.RL Ohm  g=1e-9 1/Ohm  i_specify=off  i_priority=None  i=0 A  i_nominal_specify=off  i_nominal_value=1  i_nominal_unit=A  v_specify=off  v_priority=None  v=0 V  v_nominal_specify=off  v_nominal_value=1  v_nominal_unit=V  i_L_specify=on  i_L_priority=High  i_L=0 A  i_L_nominal_specify=off  i_L_nominal_value=1  i_L_nominal_unit=A
  R_misc : fl_lib/Electrical/Electrical Elements/Resistor  R=TB.A.Rmisc Ohm  i_specify=off  i_priority=None  i=0 A  i_nominal_specify=off  i_nominal_value=1  i_nominal_unit=A  v_specify=off  v_priority=None  v=0 V  v_nominal_specify=off  v_nominal_value=1  v_nominal_unit=V
  S1_VIN_A : Subsystem  mask(PRISM-Hub switch cell){Ron=TB.A.Rds, Goff=TB.A.Goff, Vf=TB.A.Vf, Rd=TB.A.Rd, Goffd=TB.A.Goffd}
      mask prompts: Ron "도통 저항 R_on [Ohm]"; Goff "차단 컨덕턴스 G_off [S]"; Vf "다이오드 순방향 전압 Vf [V]"; Rd "다이오드 도통 저항 R_d [Ohm]"; Goffd "다이오드 차단 컨덕턴스 [S]"
      mask help: 전력 반도체 스위치 셀 S1. 게이트 태그 gA_P3_S1.
      settings: AttributesFormatString=gate: gA_P3_S1
      mask Display:
      | plot([0.05 0.35 ],[0.50 0.50 ],[0.35 0.65 ],[0.50 0.74 ],[0.65 0.95 ],[0.50 0.50 ]);
      | plot([0.20 0.20 0.42 ],[0.50 0.20 0.20 ],[0.58 0.80 0.80 ],[0.20 0.20 0.50 ]);
      | plot([0.42 0.58 0.58 0.42 ],[0.20 0.10 0.30 0.20 ],[0.42 0.42 ],[0.10 0.30 ]);
      | text(0.5,0.80,'S1','horizontalAlignment','center','texmode','off');
      | port_label('LConn',1,'D');
      | port_label('RConn',1,'S');
  S2_A_VOUT : Subsystem  mask(PRISM-Hub switch cell){Ron=TB.A.Rds, Goff=TB.A.Goff, Vf=TB.A.Vf, Rd=TB.A.Rd, Goffd=TB.A.Goffd}
      mask prompts: Ron "도통 저항 R_on [Ohm]"; Goff "차단 컨덕턴스 G_off [S]"; Vf "다이오드 순방향 전압 Vf [V]"; Rd "다이오드 도통 저항 R_d [Ohm]"; Goffd "다이오드 차단 컨덕턴스 [S]"
      mask help: 전력 반도체 스위치 셀 S2. 게이트 태그 gA_P3_S2.
      settings: AttributesFormatString=gate: gA_P3_S2
      mask Display:
      | plot([0.05 0.35 ],[0.50 0.50 ],[0.35 0.65 ],[0.50 0.74 ],[0.65 0.95 ],[0.50 0.50 ]);
      | plot([0.20 0.20 0.42 ],[0.50 0.20 0.20 ],[0.58 0.80 0.80 ],[0.20 0.20 0.50 ]);
      | plot([0.42 0.58 0.58 0.42 ],[0.20 0.10 0.30 0.20 ],[0.42 0.42 ],[0.10 0.30 ]);
      | text(0.5,0.80,'S2','horizontalAlignment','center','texmode','off');
      | port_label('LConn',1,'D');
      | port_label('RConn',1,'S');
  S3_VOUT_B : Subsystem  mask(PRISM-Hub switch cell){Ron=TB.A.Rds, Goff=TB.A.Goff, Vf=TB.A.Vf, Rd=TB.A.Rd, Goffd=TB.A.Goffd}
      mask prompts: Ron "도통 저항 R_on [Ohm]"; Goff "차단 컨덕턴스 G_off [S]"; Vf "다이오드 순방향 전압 Vf [V]"; Rd "다이오드 도통 저항 R_d [Ohm]"; Goffd "다이오드 차단 컨덕턴스 [S]"
      mask help: 전력 반도체 스위치 셀 S3. 게이트 태그 gA_P3_S3.
      settings: AttributesFormatString=gate: gA_P3_S3
      mask Display:
      | plot([0.95 0.65 ],[0.50 0.50 ],[0.65 0.35 ],[0.50 0.74 ],[0.35 0.05 ],[0.50 0.50 ]);
      | plot([0.80 0.80 0.58 ],[0.50 0.20 0.20 ],[0.42 0.20 0.20 ],[0.20 0.20 0.50 ]);
      | plot([0.58 0.42 0.42 0.58 ],[0.20 0.10 0.30 0.20 ],[0.58 0.58 ],[0.10 0.30 ]);
      | text(0.5,0.80,'S3','horizontalAlignment','center','texmode','off');
      | port_label('LConn',1,'D');
      | port_label('RConn',1,'S');
  S4_B_GND : Subsystem  mask(PRISM-Hub switch cell){Ron=TB.A.Rds, Goff=TB.A.Goff, Vf=TB.A.Vf, Rd=TB.A.Rd, Goffd=TB.A.Goffd}
      mask prompts: Ron "도통 저항 R_on [Ohm]"; Goff "차단 컨덕턴스 G_off [S]"; Vf "다이오드 순방향 전압 Vf [V]"; Rd "다이오드 도통 저항 R_d [Ohm]"; Goffd "다이오드 차단 컨덕턴스 [S]"
      mask help: 전력 반도체 스위치 셀 S4. 게이트 태그 gA_P3_S4.
      settings: AttributesFormatString=gate: gA_P3_S4
      mask Display:
      | plot([0.95 0.65 ],[0.50 0.50 ],[0.65 0.35 ],[0.50 0.74 ],[0.35 0.05 ],[0.50 0.50 ]);
      | plot([0.80 0.80 0.58 ],[0.50 0.20 0.20 ],[0.42 0.20 0.20 ],[0.20 0.20 0.50 ]);
      | plot([0.58 0.42 0.42 0.58 ],[0.20 0.10 0.30 0.20 ],[0.58 0.58 ],[0.10 0.30 ]);
      | text(0.5,0.80,'S4','horizontalAlignment','center','texmode','off');
      | port_label('LConn',1,'D');
      | port_label('RConn',1,'S');
  V_Cfly : fl_lib/Electrical/Electrical Sensors/Voltage Sensor
  iA_P3_PS2SL : nesl_utility/PS-Simulink Converter  PhysicalDomain=network_engine_domain  SubClassName=ps_output  LeftPortType=input  RightPortType=output  PseudoPeriodic=off  Frequencies=[]  VectorFormat=inherit  Unit=inherit  AffineConversion=off
  vCf_P3_PS2SL : nesl_utility/PS-Simulink Converter  PhysicalDomain=network_engine_domain  SubClassName=ps_output  LeftPortType=input  RightPortType=output  PseudoPeriodic=off  Frequencies=[]  VectorFormat=inherit  Unit=inherit  AffineConversion=off
  VIN : PMIOPort  Side=Left
  GND : PMIOPort  Port=2  Side=Left
  VOUT : PMIOPort  Port=3  Side=Right
  tag scope: iA_P3=global, vCf_P3=global
  wires:
  iA_P3_PS2SL/1 -> [iA_P3]
  vCf_P3_PS2SL/1 -> [vCf_P3]
  connections:
  VIN/RConn1 -- S1_VIN_A/LConn1
  S2_A_VOUT/LConn1 -- S1_VIN_A/RConn1 -- R_misc/LConn1
  R_misc/RConn1 -- L_r/LConn1
  L_r/RConn1 -- I_Cfly/LConn1
  C_fly/LConn1 -- I_Cfly/RConn2 -- V_Cfly/LConn1
  S4_B_GND/LConn1 -- C_fly/RConn1 -- S3_VOUT_B/RConn1 -- V_Cfly/RConn2
  S4_B_GND/RConn1 -- GND/RConn1
  VOUT/RConn1 -- S2_A_VOUT/RConn1 -- S3_VOUT_B/LConn1
  I_Cfly/RConn1 -- iA_P3_PS2SL/LConn1
  V_Cfly/RConn1 -- vCf_P3_PS2SL/LConn1

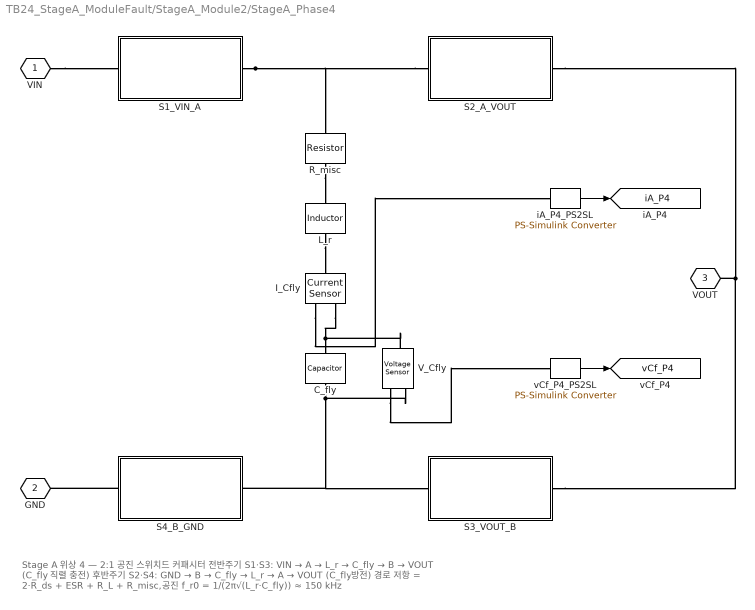
== system TB24_StageA_ModuleFault/StageA_Module2/StageA_Phase4 ==
  note: Stage A 위상 4 — 2:1 공진 스위치드 커패시터
      | 전반주기 S1·S3: VIN → A → L_r → C_fly → B → VOUT (C_fly 직렬 충전)
      | 후반주기 S2·S4: GND → B → C_fly → L_r → A → VOUT (C_fly 방전)
      | 경로 저항 = 2·R_ds + ESR + R_L + R_misc, 공진 f_r0 = 1/(2π√(L_r·C_fly)) ≈ 150 kHz
  C_fly : fl_lib/Electrical/Electrical Elements/Capacitor  c=TB.A.Cfly F  r=TB.A.ESR Ohm  g=0 1/Ohm  i_specify=off  i_priority=None  i=0 A  i_nominal_specify=off  i_nominal_value=1  i_nominal_unit=A  v_specify=off  v_priority=None  v=0 V  v_nominal_specify=off  v_nominal_value=1  v_nominal_unit=V  vc_specify=on  vc_priority=High  vc=TB.vC0_ph(4) V  vc_nominal_specify=off  vc_nominal_value=1  vc_nominal_unit=V
  I_Cfly : fl_lib/Electrical/Electrical Sensors/Current Sensor
  L_r : fl_lib/Electrical/Electrical Elements/Inductor  l=TB.A.Lr H  r=TB.A.RL Ohm  g=1e-9 1/Ohm  i_specify=off  i_priority=None  i=0 A  i_nominal_specify=off  i_nominal_value=1  i_nominal_unit=A  v_specify=off  v_priority=None  v=0 V  v_nominal_specify=off  v_nominal_value=1  v_nominal_unit=V  i_L_specify=on  i_L_priority=High  i_L=0 A  i_L_nominal_specify=off  i_L_nominal_value=1  i_L_nominal_unit=A
  R_misc : fl_lib/Electrical/Electrical Elements/Resistor  R=TB.A.Rmisc Ohm  i_specify=off  i_priority=None  i=0 A  i_nominal_specify=off  i_nominal_value=1  i_nominal_unit=A  v_specify=off  v_priority=None  v=0 V  v_nominal_specify=off  v_nominal_value=1  v_nominal_unit=V
  S1_VIN_A : Subsystem  mask(PRISM-Hub switch cell){Ron=TB.A.Rds, Goff=TB.A.Goff, Vf=TB.A.Vf, Rd=TB.A.Rd, Goffd=TB.A.Goffd}
      mask prompts: Ron "도통 저항 R_on [Ohm]"; Goff "차단 컨덕턴스 G_off [S]"; Vf "다이오드 순방향 전압 Vf [V]"; Rd "다이오드 도통 저항 R_d [Ohm]"; Goffd "다이오드 차단 컨덕턴스 [S]"
      mask help: 전력 반도체 스위치 셀 S1. 게이트 태그 gA_P4_S1.
      settings: AttributesFormatString=gate: gA_P4_S1
      mask Display:
      | plot([0.05 0.35 ],[0.50 0.50 ],[0.35 0.65 ],[0.50 0.74 ],[0.65 0.95 ],[0.50 0.50 ]);
      | plot([0.20 0.20 0.42 ],[0.50 0.20 0.20 ],[0.58 0.80 0.80 ],[0.20 0.20 0.50 ]);
      | plot([0.42 0.58 0.58 0.42 ],[0.20 0.10 0.30 0.20 ],[0.42 0.42 ],[0.10 0.30 ]);
      | text(0.5,0.80,'S1','horizontalAlignment','center','texmode','off');
      | port_label('LConn',1,'D');
      | port_label('RConn',1,'S');
  S2_A_VOUT : Subsystem  mask(PRISM-Hub switch cell){Ron=TB.A.Rds, Goff=TB.A.Goff, Vf=TB.A.Vf, Rd=TB.A.Rd, Goffd=TB.A.Goffd}
      mask prompts: Ron "도통 저항 R_on [Ohm]"; Goff "차단 컨덕턴스 G_off [S]"; Vf "다이오드 순방향 전압 Vf [V]"; Rd "다이오드 도통 저항 R_d [Ohm]"; Goffd "다이오드 차단 컨덕턴스 [S]"
      mask help: 전력 반도체 스위치 셀 S2. 게이트 태그 gA_P4_S2.
      settings: AttributesFormatString=gate: gA_P4_S2
      mask Display:
      | plot([0.05 0.35 ],[0.50 0.50 ],[0.35 0.65 ],[0.50 0.74 ],[0.65 0.95 ],[0.50 0.50 ]);
      | plot([0.20 0.20 0.42 ],[0.50 0.20 0.20 ],[0.58 0.80 0.80 ],[0.20 0.20 0.50 ]);
      | plot([0.42 0.58 0.58 0.42 ],[0.20 0.10 0.30 0.20 ],[0.42 0.42 ],[0.10 0.30 ]);
      | text(0.5,0.80,'S2','horizontalAlignment','center','texmode','off');
      | port_label('LConn',1,'D');
      | port_label('RConn',1,'S');
  S3_VOUT_B : Subsystem  mask(PRISM-Hub switch cell){Ron=TB.A.Rds, Goff=TB.A.Goff, Vf=TB.A.Vf, Rd=TB.A.Rd, Goffd=TB.A.Goffd}
      mask prompts: Ron "도통 저항 R_on [Ohm]"; Goff "차단 컨덕턴스 G_off [S]"; Vf "다이오드 순방향 전압 Vf [V]"; Rd "다이오드 도통 저항 R_d [Ohm]"; Goffd "다이오드 차단 컨덕턴스 [S]"
      mask help: 전력 반도체 스위치 셀 S3. 게이트 태그 gA_P4_S3.
      settings: AttributesFormatString=gate: gA_P4_S3
      mask Display:
      | plot([0.95 0.65 ],[0.50 0.50 ],[0.65 0.35 ],[0.50 0.74 ],[0.35 0.05 ],[0.50 0.50 ]);
      | plot([0.80 0.80 0.58 ],[0.50 0.20 0.20 ],[0.42 0.20 0.20 ],[0.20 0.20 0.50 ]);
      | plot([0.58 0.42 0.42 0.58 ],[0.20 0.10 0.30 0.20 ],[0.58 0.58 ],[0.10 0.30 ]);
      | text(0.5,0.80,'S3','horizontalAlignment','center','texmode','off');
      | port_label('LConn',1,'D');
      | port_label('RConn',1,'S');
  S4_B_GND : Subsystem  mask(PRISM-Hub switch cell){Ron=TB.A.Rds, Goff=TB.A.Goff, Vf=TB.A.Vf, Rd=TB.A.Rd, Goffd=TB.A.Goffd}
      mask prompts: Ron "도통 저항 R_on [Ohm]"; Goff "차단 컨덕턴스 G_off [S]"; Vf "다이오드 순방향 전압 Vf [V]"; Rd "다이오드 도통 저항 R_d [Ohm]"; Goffd "다이오드 차단 컨덕턴스 [S]"
      mask help: 전력 반도체 스위치 셀 S4. 게이트 태그 gA_P4_S4.
      settings: AttributesFormatString=gate: gA_P4_S4
      mask Display:
      | plot([0.95 0.65 ],[0.50 0.50 ],[0.65 0.35 ],[0.50 0.74 ],[0.35 0.05 ],[0.50 0.50 ]);
      | plot([0.80 0.80 0.58 ],[0.50 0.20 0.20 ],[0.42 0.20 0.20 ],[0.20 0.20 0.50 ]);
      | plot([0.58 0.42 0.42 0.58 ],[0.20 0.10 0.30 0.20 ],[0.58 0.58 ],[0.10 0.30 ]);
      | text(0.5,0.80,'S4','horizontalAlignment','center','texmode','off');
      | port_label('LConn',1,'D');
      | port_label('RConn',1,'S');
  V_Cfly : fl_lib/Electrical/Electrical Sensors/Voltage Sensor
  iA_P4_PS2SL : nesl_utility/PS-Simulink Converter  PhysicalDomain=network_engine_domain  SubClassName=ps_output  LeftPortType=input  RightPortType=output  PseudoPeriodic=off  Frequencies=[]  VectorFormat=inherit  Unit=inherit  AffineConversion=off
  vCf_P4_PS2SL : nesl_utility/PS-Simulink Converter  PhysicalDomain=network_engine_domain  SubClassName=ps_output  LeftPortType=input  RightPortType=output  PseudoPeriodic=off  Frequencies=[]  VectorFormat=inherit  Unit=inherit  AffineConversion=off
  VIN : PMIOPort  Side=Left
  GND : PMIOPort  Port=2  Side=Left
  VOUT : PMIOPort  Port=3  Side=Right
  tag scope: iA_P4=global, vCf_P4=global
  wires:
  iA_P4_PS2SL/1 -> [iA_P4]
  vCf_P4_PS2SL/1 -> [vCf_P4]
  connections:
  VIN/RConn1 -- S1_VIN_A/LConn1
  S2_A_VOUT/LConn1 -- S1_VIN_A/RConn1 -- R_misc/LConn1
  R_misc/RConn1 -- L_r/LConn1
  L_r/RConn1 -- I_Cfly/LConn1
  C_fly/LConn1 -- I_Cfly/RConn2 -- V_Cfly/LConn1
  S4_B_GND/LConn1 -- C_fly/RConn1 -- S3_VOUT_B/RConn1 -- V_Cfly/RConn2
  S4_B_GND/RConn1 -- GND/RConn1
  VOUT/RConn1 -- S2_A_VOUT/RConn1 -- S3_VOUT_B/LConn1
  I_Cfly/RConn1 -- iA_P4_PS2SL/LConn1
  V_Cfly/RConn1 -- vCf_P4_PS2SL/LConn1
